simulink model "Sim_PMSMCtrl"  (R2025b)
settings: Solver=FixedStepAuto  StartTime=0.0  StopTime=0.1  RelTol=1e-3
values from neighbouring files (symbols this model uses):
  Par_Sim_cdSysTs = 5.0E-8    [Sim_PMSMCtrl.sldd]
undefined symbols (not defined in the file or in its folder): Par_Cpu_cfCoreFrc, Par_Cpu_cfTpwm
libraries: nesl_utility x14, fl_lib x8, ee_lib x5, mcbeeMathTransformLib x4, Lib_General x3, batteryecm_lib x1, Lib_PMSMCtrl x1
settings Model: DataDictionary=Sim_PMSMCtrl.sldd  SimulationMode=accelerator  Creator=62555  LastModifiedBy=62555
settings OptimizationCC: DefaultParameterBehavior=Inlined  UseDivisionForNetSlopeComputation=on  DefaultUnderspecifiedDataType=single  EnhancedBackFolding=on  PassReuseOutputArgsAs=Individual arguments  ZeroExternalMemoryAtStartup=off  ZeroInternalMemoryAtStartup=off  OptimizeBlockOrder=speed  DifferentSizesBufferReuse=on  OptimizationCustomize=off  EfficientTunableParamExpr=on
settings DebuggingCC: ParameterPrecisionLossMsg=none  ParameterTunabilityLossMsg=error
settings SFSimCC: MATLABDynamicMemAlloc=off
settings RTWCC: SystemTargetFile=ert.tlc  GenCodeOnly=on  TemplateMakefile=ert_default_tmf  GenerateReport=on  Toolchain=CMake  LaunchReport=on  GPUComputeCapability=3.5  Description=Embedded Coder
settings CodeAppCC: ForceParamTrailComments=on  IgnoreCustomStorageClasses=off  OperatorAnnotations=on  SimulinkDataObjDesc=on  SFDataObjDesc=on  InsertBlockDesc=on
settings ERTTargetCC: ERTCustomFileTemplate=example_file_process.tlc  DynamicArrayContainerType=coder::array  TargetLangStandard=C99 (ISO)  GenerateSampleERTMain=on

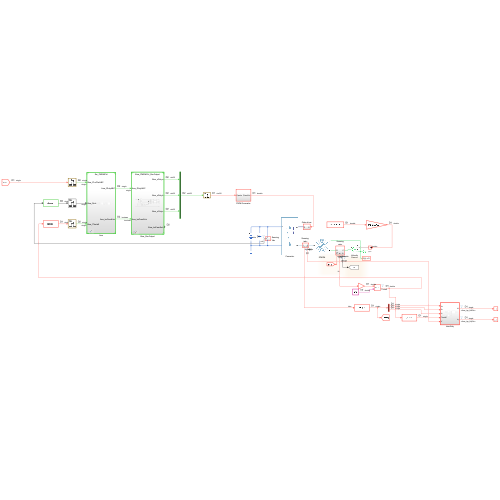
[thumbnail: Simulink's stored preview of the top-level diagram]
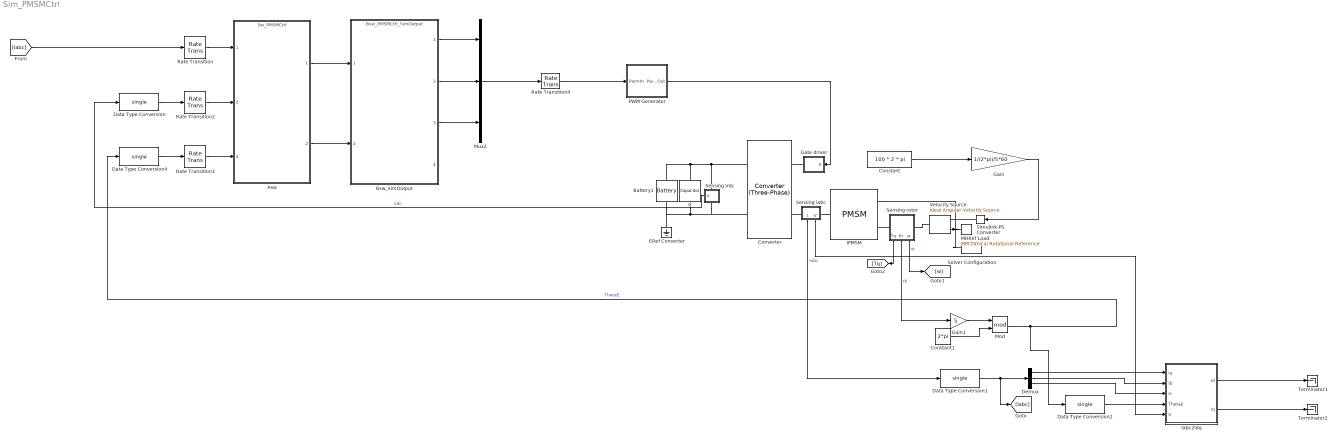
== system Sim_PMSMCtrl ==
  Asw : ModelReference  ModelNameDialog=Sw_PMSMCtrl.slx  SimulationMode=Normal  ModelReferenceVersion=6.16
  Battery1 : batteryecm_lib/Battery  Vnom=48 V  prm_dir=1  R1_dis=2 Ohm  R1_ch=2 Ohm  R1=0.001 Ohm  prm_AH=1  AH=300 hr*A  V1=V1 V  AH1=100 hr*A  prm_R2=1  R2=2000 Ohm  Tmeas=298.15 K  charge_measurement_port=simscape.enum.battery.enable.no  prm_dyn=1  Rp1=0.005 Ohm  tau1=30 s  Rp2=0.005 Ohm  tau2=30 s  Rp3=0.005 Ohm  tau3=30 s  Rp4=0.005 Ohm  tau4=30 s  Rp5=0.005 Ohm  tau5=30 s  prm_fade=1  N_fade=100  AH_fade=45 hr*A  R1_fade=2.02 Ohm  R1_ch_fade=2.02 Ohm  V1_fade=10.35 V  prm_age=1  prm_age_OCV=1  OCV_age=0.9  SOC_age=60  Tmeas_age=298.15 K  delta_time_age_vec=[0] d  temperature_age_vec=[273] K  OCV_scaling_age=2.2134e6  OCV_offset_age=1.632e6  temp_exp_age=0.515833569 V  t_exp_age=0.75  Vnom_T2=12 V  R1_T2=2.2 Ohm  R1_T2_dis=2.2 Ohm  R1_T2_ch=2.2 Ohm  V1_T2=11.4 V  R2_T2=2200 Ohm  Rp1_T2=0.005 Ohm  tau1_T2=30 s  Rp2_T2=0.005 Ohm  tau2_T2=30 s  Rp3_T2=0.005 Ohm  tau3_T2=30 s  Rp4_T2=0.005 Ohm  tau4_T2=30 s  Rp5_T2=0.005 Ohm  tau5_T2=30 s  Tmeas2=273.15 K  thermal_port=simscape.enum.thermaleffects.omit  thermal_mass=30000 J/K  i_specify=off  i_priority=None  i=0 A  i_nominal_specify=off  i_nominal_value=1  i_nominal_unit=A  v_specify=off  v_priority=None  v=0 V  v_nominal_specify=off  v_nominal_value=1  v_nominal_unit=V  charge_specify=on  charge_priority=High  charge=50 hr*A  charge_nominal_specify=off  charge_nominal_value=1  charge_nominal_unit=A*hr  num_cycles_specify=off  num_cycles_priority=High  num_cycles=0  num_cycles_nominal_specify=off  num_cycles_nominal_value=1  num_cycles_nominal_unit=1  temperature_specify=off  temperature_priority=High  temperature=298.15 K  temperature_nominal_specify=off  temperature_nominal_value=1  temperature_nominal_unit=K
  Bsw_SimOutput : ModelReference  ModelNameDialog=Bsw_PMSMCtrl_SimOutput.slx  SimulationMode=Normal  ModelReferenceVersion=6.3
  C : fl_lib/Electrical/Electrical Elements/Capacitor  c=5e-6 F  r=1e-6 Ohm  g=0 1/Ohm  i_specify=off  i_priority=None  i=0 A  i_nominal_specify=off  i_nominal_value=1  i_nominal_unit=A  v_specify=off  v_priority=None  v=0 V  v_nominal_specify=off  v_nominal_value=1  v_nominal_unit=V  vc_specify=on  vc_priority=None  vc=48 V  vc_nominal_specify=off  vc_nominal_value=1  vc_nominal_unit=V
  Constant : Constant  Value=100 * 2 * pi  SampleTime=-1
  Constant1 : Constant  Value=2*pi
  Converter : ee_lib/Semiconductors & Converters/Converters/Converter (Three-Phase)  port_option=ee.enum.threePhasePort.composite  fidelity_option=ee.enum.converters.fidelity.detailed  device_type=ee.enum.converters.switchingdevice.mosfet  showThermalPort=false  K=0  Vth=0.005 V  Vgt=1 V  Vgt_off=-1 V  Ih=1 A  Vf=0.005 V  Ron=0.001 Ohm  Rds=0.001 Ohm  Goff=1e-5 1/Ohm  Eon_scalar=22.86e-3 J  Eoff_scalar=17.14e-3 J  Eoff_natural_commutation=10e-3 J  Voff=300 V  Iout_scalar=600 A  onCurrentMeasDelay=0 s  useCurrentFromPreviousCycle=false  useVoltageFromPreviousCycle=false  diode_param=ee.enum.converters.protectiondiode.none  diode_Vf=0.8 V  diode_Ron=0.001 Ohm  diode_Goff=1e-5 1/Ohm  diode_C=50 nF  diode_iRM=-235 A  diode_iF=300 A  diode_idot=-50 A/us  diode_trr_param=1  diode_trr_factor=3  diode_trr=15 us  diode_Qrr=1.5e+3 s*uA  diode_rec_loss_model=ee.enum.diode.reverseRecoveryModel.fixed  diode_ErecVal=0 J  diode_scaleWithIandV=false  diode_ErecMat=zeros(2, 3) J  diode_TjrecVec=[298.15, 398.15] K  diode_IfrecVec=[.1, 1, 10] A  diode_IrecVal=10 A  diode_VrecVal=10 V  diode_tFilter=1 / 1000 / 100 s  thermal_network_parameterization=ee.enum.thermalNetworkTopology.external  Rth=[.08, .5] K/W  Rth_Cauer=[.08, .1, .5] K/W  Rth_Foster=[.08, .14, .22, .16] K/W  thermal_mass_parameterization=ee.enum.thermalNetwork.timeconstant  thermal_mass=[.01, .5] J/K  thermal_mass_Cauer=[.01, .1, .5] J/K  thermal_mass_Foster=[.001, .005, .05, .5] J/K  thermal_time_constant=[.001, .2] s  thermal_time_constant_Cauer=[.001, .1, .2] s  thermal_time_constant_Foster=[7e-05, .0007, .01, .08] s  thermal_mass_initial_temperatures=[25, 25] degC  thermal_mass_initial_temperatures_Cauer=[25, 25, 25] degC  junction_thermal_mass=0.01 J/K  Tvec_initial_Foster=[25, 25, 25, 25] degC  snubber_type=0  Cs=1e-7 F  Rs=0.1 Ohm  Vce_loss=[0, 150, 300] V
  Data Type Conversion{,1..2,4} (4 alike) : DataTypeConversion  OutDataTypeStr=single  SaturateOnIntegerOverflow=off  RndMeth=Floor
  Demux : Demux  Outputs=3
  ERef Converter : fl_lib/Electrical/Electrical Elements/Electrical Reference
  Gain : Gain  Gain=1/(2*pi)/5*60
  Gain1 : Gain  Gain=5
  Gate driver : Subsystem
  IPMSM : ee_lib/Electromechanical/Permanent Magnet/PMSM  port_option=ee.enum.threePhasePort.composite  winding_type=ee.enum.statorconnection.wye  machine_param=ee.enum.pmsm.parameterization.constant  nPolePairs=5  pmflux_param=ee.enum.pmflux.fluxlinkage  pm_flux_linkage=Par_Mtr_cfFlux Wb  torque_constant=0.18 N*m/A  back_emf_constant=0.18 V/(rad/s)  stator_param=ee.enum.statorparam.LdLqL0  Ld=Par_Mtr_cfLd H  Lq=Par_Mtr_cfLq H  idVec=[-200, 0, 200] A  iqVec=[-200, 0, 200] A  LdMatrix=0.0002 * ones(3, 3) H  LqMatrix=0.0002 * ones(3, 3) H  PmMatrix=0.1 * ones(3, 3) Wb  ktMatrix=0.18 * ones(3, 3) N*m/A  keMatrix=0.18 * ones(3, 3) V/(rad/s)  L0=L0 H  Ls=0.0002 H  Lm=0.00002 H  Ms=0.00002 H  Rs=Par_Mtr_cfRs Ohm  zero_sequence=ee.enum.park.zerosequence.exclude  axes_param=ee.enum.rotorangle.daxis  loss_param=ee.enum.ironloss.none  losses_oc=[0, 0, 0] W  losses_sc=[0, 0, 0] W  f_losses=60 Hz  Isc_losses=95 A  J=0 kg*m^2  lam=0 N*m/(rad/s)  i_d_specify=off  i_d_priority=None  i_d=0 A  i_d_nominal_specify=off  i_d_nominal_value=1  i_d_nominal_unit=A  i_q_specify=off  i_q_priority=None  i_q=0 A  i_q_nominal_specify=off  i_q_nominal_value=1  i_q_nominal_unit=A  torque_specify=off  torque_priority=None  torque=0 N*m  torque_nominal_specify=off  torque_nominal_value=1  torque_nominal_unit=N*m  angular_velocity_specify=on  angular_velocity_priority=None  angular_velocity=0 rad/s  angular_velocity_nominal_specify=off  angular_velocity_nominal_value=1  angular_velocity_nominal_unit=rpm  angular_position_specify=on  angular_position_priority=High  angular_position=0 rad  angular_position_nominal_specify=off  angular_position_nominal_value=1  angular_position_nominal_unit=deg  alpha=3.93e-3 1/K  alpha_flux=-0.001 1/K  Tmeas=298.15 K  stator_thermal_mass=100 J/K  rotor_thermal_mass=200 J/K  Rm_percent_rotor=90  Rd_percent_rotor=30  temperatureA_specify=off  temperatureA_priority=High  temperatureA=25 degC  temperatureA_nominal_specify=off  temperatureA_nominal_value=1  temperatureA_nominal_unit=degC  temperatureB_specify=off  temperatureB_priority=High  temperatureB=25 degC  temperatureB_nominal_specify=off  temperatureB_nominal_value=1  temperatureB_nominal_unit=degC  temperatureC_specify=off  temperatureC_priority=High  temperatureC=25 degC  temperatureC_nominal_specify=off  temperatureC_nominal_value=1  temperatureC_nominal_unit=degC  temperatureR_specify=off  temperatureR_priority=High  temperatureR=25 degC  temperatureR_nominal_specify=off  temperatureR_nominal_value=1  temperatureR_nominal_unit=degC
      settings: InternalSimscapePortConfiguration="{\"Bottom\":[],\"Left\":[{\"id\":\"N\",\"label\":\"~\",\"type\":\"foundation.electrical.three_phase\"}],\"Right\":[{\"id\":\"R\",\"label\":\"R\",\"type\":\"foundation.mechanical.rotational.rotational\"},{\"id\":\"C\",\"label\":\"C\",\"type\":\"foundation.mechanical.rotational.rotational\"}],\"Top\":[]}"
  Iabc2Idq : Subsystem  TreatAsAtomicUnit=on
      settings: RTWSystemCode=Nonreusable function  RTWFcnNameOpts=Use subsystem name  FunctionInterfaceSpec=Allow arguments (Optimized)
  MRRef Load : fl_lib/Mechanical/Rotational Elements/Mechanical Rotational Reference
  Mod : Math  Operator=mod
  Mux2 : Mux  Inputs=3
  PWM Generator : Subsystem
  Rate Transition : RateTransition  OutPortSampleTime=Par_Sw_cdTs
  Rate Transition1 : RateTransition  OutPortSampleTime=Par_Sw_cdTs
  Rate Transition2 : RateTransition  OutPortSampleTime=Par_Sw_cdTs
  Rate Transition4 : RateTransition  OutPortSampleTime=Par_Sim_cdSysTs
  Sensing Vdc : Subsystem
      settings: PortSchema="{\"entries\":[{\"content\":{\"sides\":[{\"content\":{\"connectorIds\":[\"LConn1\"]},\"type\":\"ConnectorPlacement.EquallySpacedRectSide\",\"uuid\":\"bc3757cc-4537-444e-89af-7b7d8c8c1fa7\"},{\"content\":{\"connectorIds\":[\"RConn1\"],\"side\":\"RIGHT\"},\"type\":\"ConnectorPlacement.EquallySpacedRectSide\",\"uuid\":\"908bf4c4-26f6-4d8a-bcf8-68236027f5f8\"},{\"content\":{\"connectorIds\":[\"Out1\"],\"side\":\"TOP\"},\"type\":\"ConnectorPlacement.EquallySpacedRectSide\",\"uuid\":\"33f228db-ba47-4718-96dc-a72de309ae8c\"},{\"content\":{\"connectorIds\":[],\"side\":\"BOTTOM\"},\"type\":\"ConnectorPlacement.EquallySpacedRectSide\",\"uuid\":\"d9b66c7e-0954-4c47-8bcc-77bf13ff573c\"}]},\"type\":\"ConnectorPlacement.EquallySpacedConnector\",\"uuid\":\"345f3578-0572-4e64-b2f3-84728129a12d\"}],\"packageUris\":[\"http://schema.mathworks.com/mf0/Connector/R2020b\"],\"version\":\"1.0\"}"
  Sensing rotor : Subsystem
      settings: PortSchema="{\"entries\":[{\"content\":{\"sides\":[{\"content\":{\"connectorIds\":[\"LConn1\"]},\"type\":\"ConnectorPlacement.EquallySpacedRectSide\",\"uuid\":\"bc3757cc-4537-444e-89af-7b7d8c8c1fa7\"},{\"content\":{\"connectorIds\":[\"RConn1\"],\"side\":\"RIGHT\"},\"type\":\"ConnectorPlacement.EquallySpacedRectSide\",\"uuid\":\"908bf4c4-26f6-4d8a-bcf8-68236027f5f8\"},{\"content\":{\"connectorIds\":[],\"side\":\"TOP\"},\"type\":\"ConnectorPlacement.EquallySpacedRectSide\",\"uuid\":\"33f228db-ba47-4718-96dc-a72de309ae8c\"},{\"content\":{\"connectorIds\":[\"Out1\",\"Out2\",\"Out3\"],\"side\":\"BOTTOM\"},\"type\":\"ConnectorPlacement.EquallySpacedRectSide\",\"uuid\":\"5b763560-fcc9-460b-9ba7-46235112184c\"}]},\"type\":\"ConnectorPlacement.EquallySpacedConnector\",\"uuid\":\"345f3578-0572-4e64-b2f3-84728129a12d\"}],\"packageUris\":[\"http://schema.mathworks.com/mf0/Connector/R2020b\"],\"version\":\"1.0\"}"
  Sensing iabc : Subsystem
      settings: PortSchema="{\"entries\":[{\"content\":{\"sides\":[{\"content\":{\"connectorIds\":[\"LConn1\"]},\"type\":\"ConnectorPlacement.EquallySpacedRectSide\",\"uuid\":\"bc3757cc-4537-444e-89af-7b7d8c8c1fa7\"},{\"content\":{\"connectorIds\":[\"RConn1\"],\"side\":\"RIGHT\"},\"type\":\"ConnectorPlacement.EquallySpacedRectSide\",\"uuid\":\"908bf4c4-26f6-4d8a-bcf8-68236027f5f8\"},{\"content\":{\"side\":\"TOP\"},\"type\":\"ConnectorPlacement.EquallySpacedRectSide\",\"uuid\":\"33f228db-ba47-4718-96dc-a72de309ae8c\"},{\"content\":{\"connectorIds\":[\"Out1\",\"Out2\"],\"side\":\"BOTTOM\"},\"type\":\"ConnectorPlacement.EquallySpacedRectSide\",\"uuid\":\"3b1d40a5-3c80-431c-8111-df754e0c502b\"}]},\"type\":\"ConnectorPlacement.EquallySpacedConnector\",\"uuid\":\"345f3578-0572-4e64-b2f3-84728129a12d\"}],\"packageUris\":[\"http://schema.mathworks.com/mf0/Connector/R2020b\"],\"version\":\"1.0\"}"
  Simulink-PS Converter : nesl_utility/Simulink-PS Converter  PhysicalDomain=network_engine_domain  SubClassName=ps_input  LeftPortType=input  RightPortType=output  PseudoPeriodic=off  Frequencies=[]  NoiseDistribution=none  NoiseParameters=[]  Unit=rpm  AffineConversion=off  FilteringAndDerivatives=zero  SimscapeFilterOrder=1  InputFilterTimeConstant=0.001  UdotUserProvided=1
  Solver Configuration : nesl_utility/Solver Configuration  PhysicalDomain=network_engine_domain  SubClassName=solver  LeftPortType=input  RightPortType=generic  Tones=[]  Harmonics=[]  SimulateNoise=off  Profile=off  UseLocalSampling=off  EnableSwitchedLinearOptims=on  FrequencyDomain=off  UseCCode=off  RelTol=0.001  AbsTol=1e-06  MinStep=1e-09  ToWorkspace=off  RevertToSquareIcSolve=off  NumHomotopyIterations=100  PhasorMode=off  PhasorModeNumHarmonics=1  ConsistencySolver=NEWTON_FTOL  IndexReductionMethod=DerivativeReplacement  DoDC=off  ResidualTolerance=1e-9  ConsistencyTolSource=GLOBAL  ConsistencyAbsTol=0.001  ConsistencyRelTol=0.001  ConsistencyTolFactor=0.001  UseLocalSolver=on  LocalSolverChoice=NE_BACKWARD_EULER_ADVANCER  ResolveIndetEquations=on  FunctionEvalNumThread=1  LocalSolverSampleTime=Par_Sim_cdSysTs  DoFixedCost=on  MaxNonlinIter=5  MaxModeIter=2  ComputeImpulses=off  ImpulseIterations=2  LinearAlgebra=auto  LinearAlgebraNumThread=0  EquationFormulation=NE_TIME_EF  DelaysMemoryBudget=1024  AutomaticFiltering=on  FilteringTimeConstant=0.001  PartitionStorageMethod=AS_NEEDED  PartitionMemoryBudget=1024  PartitionMethod=FAST  MultibodyUseLocalSolver=off  MultibodyLocalSolverChoice=ODE1  MultibodyLocalSolverSampleTime=0.001
  Terminator1 : Terminator
  Terminator2 : Terminator
  Velocity Source : fl_lib/Mechanical/Mechanical Sources/Ideal Angular Velocity Source
  wires:
  Rate Transition4/1 -> PWM Generator/1(PwmIn)
  Mux2/1 -> Rate Transition4/1
  Data Type Conversion4/1 -> Rate Transition1/1
  Data Type Conversion/1 -> Rate Transition2/1
  Asw/1 -> Bsw_SimOutput/1
  Bsw_SimOutput/1 -> Mux2/1
  Bsw_SimOutput/2 -> Mux2/2
  Bsw_SimOutput/3 -> Mux2/3
  Sensing Vdc/1(V) -> Data Type Conversion/1  "vdc"
  Constant/1 -> Gain/1
  Sensing iabc/1(I) -> Data Type Conversion1/1  "Iabc"
  PWM Generator/1(PwmOut) -> Gate driver/1(S)
  Sensing rotor/2(th) -> Gain1/1  "th"
  Sensing rotor/1(Tq) -> [Tq]
  Gain/1 -> Simulink-PS Converter/1
  Gain1/1 -> Mod/1
  Constant1/1 -> Mod/2
  Mod/1 -> Data Type Conversion4/1, Data Type Conversion2/1  "ThetaE"
  Demux/1 -> Iabc2Idq/1(Ia)
  Demux/2 -> Iabc2Idq/2(Ib)
  Demux/3 -> Iabc2Idq/3(Ic)
  Iabc2Idq/1(Id) -> Terminator1/1
  Iabc2Idq/2(Iq) -> Terminator2/1
  Data Type Conversion1/1 -> [Iabc], Demux/1
  Data Type Conversion2/1 -> Iabc2Idq/4(ThetaE)
  Sensing iabc/2(V) -> Iabc2Idq/5(V)
  [Iabc] -> Rate Transition/1
  Asw/2 -> Bsw_SimOutput/2
  Rate Transition/1 -> Asw/1
  Rate Transition1/1 -> Asw/3
  Sensing rotor/3(w) -> [w]  "w"
  Rate Transition2/1 -> Asw/2
  connections:
  C/LConn1 -- Converter/RConn1 -- Sensing Vdc/LConn1 -- Battery1/LConn1
  MRRef Load/LConn1 -- IPMSM/RConn2 -- Velocity Source/RConn2 -- Solver Configuration/RConn1
  C/RConn1 -- Converter/RConn2 -- Sensing Vdc/RConn1 -- Battery1/RConn1 -- ERef Converter/LConn1
  Simulink-PS Converter/RConn1 -- Velocity Source/RConn1
  Sensing iabc/LConn1 -- Converter/LConn2
  Sensing iabc/RConn1 -- IPMSM/LConn1
  Gate driver/RConn1 -- Converter/LConn1
  Sensing rotor/LConn1 -- IPMSM/RConn1
  Sensing rotor/RConn1 -- Velocity Source/LConn1

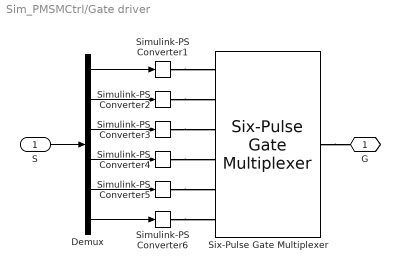
== system Sim_PMSMCtrl/Gate driver ==
  S : Inport
  Demux : Demux  Outputs=6
  Simulink-PS Converter{1..6} (6 alike) : nesl_utility/Simulink-PS Converter  PhysicalDomain=network_engine_domain  SubClassName=ps_input  LeftPortType=input  RightPortType=output  PseudoPeriodic=off  Frequencies=[]  NoiseDistribution=none  NoiseParameters=[]  Unit=1  AffineConversion=off  FilteringAndDerivatives=zero  SimscapeFilterOrder=1  InputFilterTimeConstant=0.001  UdotUserProvided=1
  Six-Pulse Gate Multiplexer : ee_lib/Semiconductors & Converters/Converters/Six-Pulse Gate Multiplexer  port_option=ee.enum.controlport.ps
  G : PMIOPort  Side=Right
  wires:
  Demux/1 -> Simulink-PS Converter1/1
  S/1 -> Demux/1
  Demux/5 -> Simulink-PS Converter5/1
  Demux/6 -> Simulink-PS Converter6/1
  Demux/4 -> Simulink-PS Converter4/1
  Demux/3 -> Simulink-PS Converter3/1
  Demux/2 -> Simulink-PS Converter2/1
  connections:
  Six-Pulse Gate Multiplexer/RConn1 -- G/RConn1
  Simulink-PS Converter1/RConn1 -- Six-Pulse Gate Multiplexer/LConn1
  Simulink-PS Converter5/RConn1 -- Six-Pulse Gate Multiplexer/LConn5
  Simulink-PS Converter6/RConn1 -- Six-Pulse Gate Multiplexer/LConn6
  Simulink-PS Converter2/RConn1 -- Six-Pulse Gate Multiplexer/LConn2
  Simulink-PS Converter3/RConn1 -- Six-Pulse Gate Multiplexer/LConn3
  Simulink-PS Converter4/RConn1 -- Six-Pulse Gate Multiplexer/LConn4

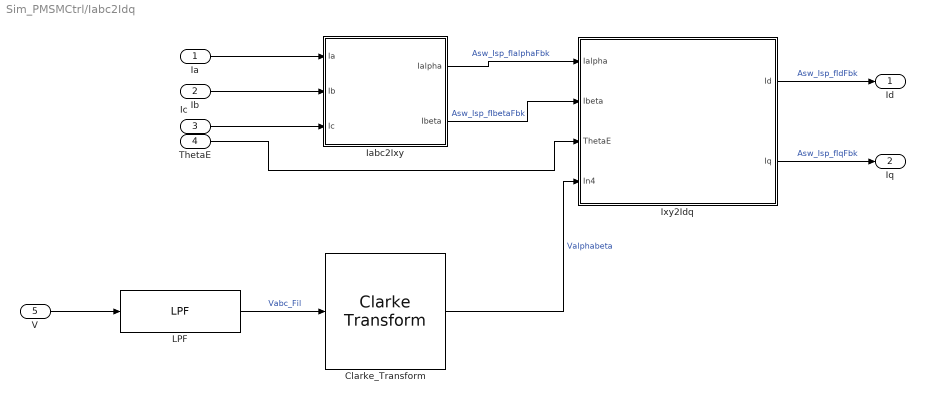
== system Sim_PMSMCtrl/Iabc2Idq ==
  Ia : Inport
  Ib : Inport  Port=2
  Ic : Inport  Port=3
  ThetaE : Inport  Port=4
  V : Inport  Port=5
  Clarke_Transform : mcbeeMathTransformLib/Clarke Transform  VariantControl=Variant2  PowerInvariant=off  UseWithEmbedded=on  PhaseInput=Three inputs
  Iabc2Ixy : Subsystem  TreatAsAtomicUnit=on
      settings: RTWSystemCode=Nonreusable function  RTWFcnNameOpts=Use subsystem name  FunctionInterfaceSpec=Allow arguments (Optimized)
  Ixy2Idq : Subsystem  TreatAsAtomicUnit=on
      settings: RTWSystemCode=Nonreusable function  RTWFcnNameOpts=Use subsystem name  FunctionInterfaceSpec=Allow arguments (Optimized)
  LPF : Lib_General/LPF  fc=1e3  Initial_condition=0  ModType=Tustin
      settings: SourceProductName=Lib_General
      settings: AttributesFormatString=|
      | fc = %<fc>
      | DisMod = %<ModType>
  Id : Outport
  Iq : Outport  Port=2
  wires:
  Ixy2Idq/2(Iq) -> Iq/1  "Asw_Isp_fIqFbk"
  Ia/1 -> Iabc2Ixy/1(Ia)
  ThetaE/1 -> Ixy2Idq/3(ThetaE)
  Ic/1 -> Iabc2Ixy/3(Ic)
  Ixy2Idq/1(Id) -> Id/1  "Asw_Isp_fIdFbk"
  Ib/1 -> Iabc2Ixy/2(Ib)
  Iabc2Ixy/2(Ibeta) -> Ixy2Idq/2(Ibeta)  "Asw_Isp_fIbetaFbk"
  Iabc2Ixy/1(Ialpha) -> Ixy2Idq/1(Ialpha)  "Asw_Isp_fIalphaFbk"
  Clarke_Transform/1 -> Ixy2Idq/4(In4)  "Valphabeta"
  V/1 -> LPF/1
  LPF/1 -> Clarke_Transform/1  "Vabc_Fil"

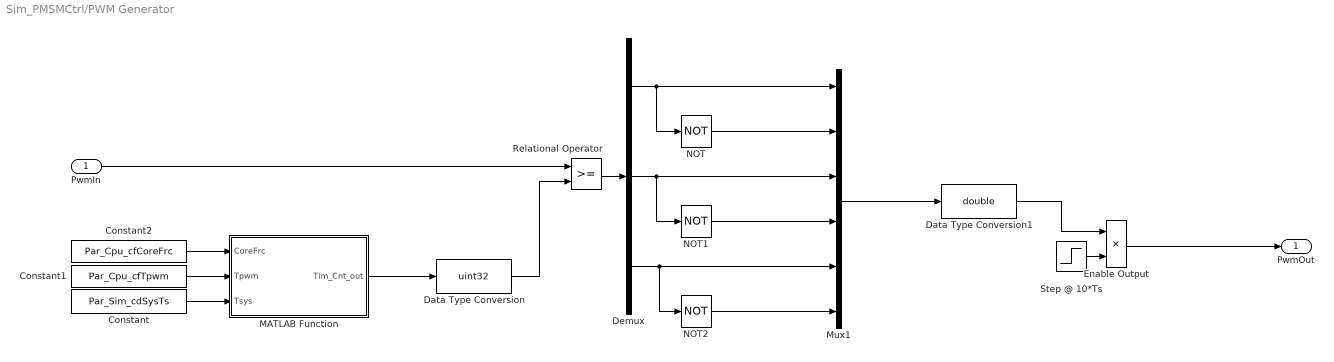
== system Sim_PMSMCtrl/PWM Generator ==
  PwmIn : Inport
  Constant : Constant  Value=Par_Sim_cdSysTs  OutDataTypeStr=double  SampleTime=-1
  Constant1 : Constant  Value=Par_Cpu_cfTpwm  OutDataTypeStr=double  SampleTime=-1
  Constant2 : Constant  Value=Par_Cpu_cfCoreFrc  OutDataTypeStr=double  SampleTime=-1
  Data Type Conversion : DataTypeConversion  OutDataTypeStr=uint32  SaturateOnIntegerOverflow=off  RndMeth=Floor
  Data Type Conversion1 : DataTypeConversion  OutDataTypeStr=double  SaturateOnIntegerOverflow=off  RndMeth=Floor
  Demux : Demux  Outputs=3
  Enable Output : Product
  MATLAB Function : MATLAB Function  TreatAsAtomicUnit=on
  Mux1 : Mux  Inputs=6
  NOT : Logic  Operator=NOT  IconShape=distinctive  AllPortsSameDT=off  OutDataTypeStr=boolean
  NOT1 : Logic  Operator=NOT  IconShape=distinctive  AllPortsSameDT=off  OutDataTypeStr=boolean
  NOT2 : Logic  Operator=NOT  IconShape=distinctive  AllPortsSameDT=off  OutDataTypeStr=boolean
  Relational Operator : RelationalOperator  OutDataTypeStr=boolean  RndMeth=Simplest  InputSameDT=off
  Step @ 10*Ts : Step  Time=0.00050  SampleTime=Par_Sim_cdSysTs
  PwmOut : Outport
  wires:
  Demux/1 -> Mux1/1, NOT/1
  Demux/3 -> NOT2/1, Mux1/5
  Demux/2 -> NOT1/1, Mux1/3
  NOT2/1 -> Mux1/6
  NOT/1 -> Mux1/2
  MATLAB Function/1(Tim_Cnt_out) -> Data Type Conversion/1
  NOT1/1 -> Mux1/4
  Relational Operator/1 -> Demux/1
  PwmIn/1 -> Relational Operator/1
  Constant/1 -> MATLAB Function/3(Tsys)
  Constant1/1 -> MATLAB Function/2(Tpwm)
  Constant2/1 -> MATLAB Function/1(CoreFrc)
  Data Type Conversion/1 -> Relational Operator/2
  Mux1/1 -> Data Type Conversion1/1
  Data Type Conversion1/1 -> Enable Output/1
  Step @ 10*Ts/1 -> Enable Output/2
  Enable Output/1 -> PwmOut/1

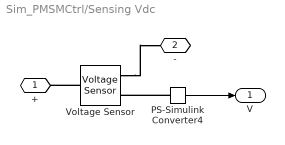
== system Sim_PMSMCtrl/Sensing Vdc ==
  PS-Simulink Converter4 : nesl_utility/PS-Simulink Converter  PhysicalDomain=network_engine_domain  SubClassName=ps_output  LeftPortType=input  RightPortType=output  PseudoPeriodic=off  Frequencies=[]  VectorFormat=1-D array  Unit=V  AffineConversion=off
  Voltage Sensor : fl_lib/Electrical/Electrical Sensors/Voltage Sensor
  + : PMIOPort  Side=Left
  - : PMIOPort  Port=2  Side=Right
  V : Outport
  wires:
  PS-Simulink Converter4/1 -> V/1
  connections:
  Voltage Sensor/LConn1 -- +/RConn1
  Voltage Sensor/RConn2 -- -/RConn1
  PS-Simulink Converter4/LConn1 -- Voltage Sensor/RConn1

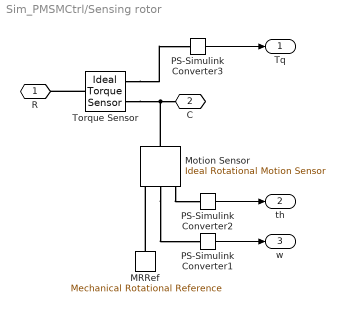
== system Sim_PMSMCtrl/Sensing rotor ==
  MRRef : fl_lib/Mechanical/Rotational Elements/Mechanical Rotational Reference
  Motion Sensor : fl_lib/Mechanical/Mechanical Sensors/Ideal Rotational Motion Sensor  reference=foundation.enum.MeasurementReference.difference  acceleration_port=false  velocity_port=true  position_port=true  wrap_angle=simscape.enum.onoff.off  offset=0 deg
  PS-Simulink Converter1 : nesl_utility/PS-Simulink Converter  PhysicalDomain=network_engine_domain  SubClassName=ps_output  LeftPortType=input  RightPortType=output  PseudoPeriodic=off  Frequencies=[]  VectorFormat=1-D array  Unit=rad/s  AffineConversion=off
  PS-Simulink Converter2 : nesl_utility/PS-Simulink Converter  PhysicalDomain=network_engine_domain  SubClassName=ps_output  LeftPortType=input  RightPortType=output  PseudoPeriodic=off  Frequencies=[]  VectorFormat=1-D array  Unit=rad  AffineConversion=off
  PS-Simulink Converter3 : nesl_utility/PS-Simulink Converter  PhysicalDomain=network_engine_domain  SubClassName=ps_output  LeftPortType=input  RightPortType=output  PseudoPeriodic=off  Frequencies=[]  VectorFormat=1-D array  Unit=N*m  AffineConversion=off
  Torque Sensor : fl_lib/Mechanical/Mechanical Sensors/Ideal Torque Sensor
  R : PMIOPort  Side=Left
  C : PMIOPort  Port=2  Side=Right
  Tq : Outport
  th : Outport  Port=2
  w : Outport  Port=3
  wires:
  PS-Simulink Converter3/1 -> Tq/1
  PS-Simulink Converter2/1 -> th/1
  PS-Simulink Converter1/1 -> w/1
  connections:
  Torque Sensor/RConn1 -- Motion Sensor/LConn1 -- C/RConn1
  Torque Sensor/RConn2 -- PS-Simulink Converter3/LConn1
  Torque Sensor/LConn1 -- R/RConn1
  Motion Sensor/RConn2 -- PS-Simulink Converter1/LConn1
  MRRef/LConn1 -- Motion Sensor/RConn1
  Motion Sensor/RConn3 -- PS-Simulink Converter2/LConn1

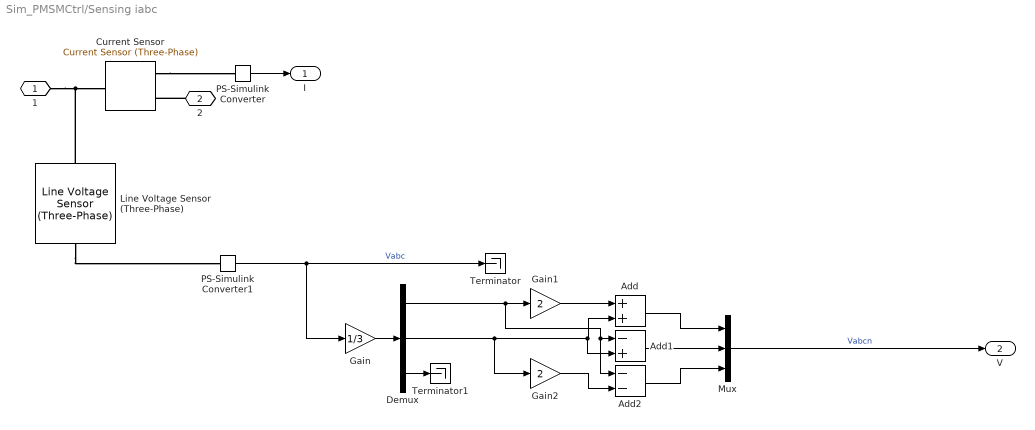
== system Sim_PMSMCtrl/Sensing iabc ==
  Add : Sum
  Add1 : Sum  Inputs=-+
  Add2 : Sum  Inputs=--
  Current Sensor : ee_lib/Sensors & Transducers/Current Sensor (Three-Phase)
  Demux : Demux  Outputs=3
  Gain : Gain  Gain=1/3
  Gain1 : Gain  Gain=2
  Gain2 : Gain  Gain=2
  Line Voltage Sensor (Three-Phase) : ee_lib/Sensors & Transducers/Line Voltage Sensor (Three-Phase)
  Mux : Mux  Inputs=3
  PS-Simulink Converter : nesl_utility/PS-Simulink Converter  PhysicalDomain=network_engine_domain  SubClassName=ps_output  LeftPortType=input  RightPortType=output  PseudoPeriodic=off  Frequencies=[]  VectorFormat=1-D array  Unit=A  AffineConversion=off
  PS-Simulink Converter1 : nesl_utility/PS-Simulink Converter  PhysicalDomain=network_engine_domain  SubClassName=ps_output  LeftPortType=input  RightPortType=output  PseudoPeriodic=off  Frequencies=[]  VectorFormat=1-D array  Unit=V  AffineConversion=off
  Terminator : Terminator
  Terminator1 : Terminator
  1 : PMIOPort  Side=Left
  2 : PMIOPort  Port=2  Side=Right
  I : Outport
  V : Outport  Port=2
  wires:
  PS-Simulink Converter/1 -> I/1
  PS-Simulink Converter1/1 -> Terminator/1, Gain/1  "Vabc"
  Gain/1 -> Demux/1
  Gain1/1 -> Add/1
  Demux/2 -> Gain2/1, Add1/2, Add/2
  Gain2/1 -> Add2/2
  Demux/1 -> Add2/1, Add1/1, Gain1/1
  Add1/1 -> Mux/2
  Add/1 -> Mux/1
  Add2/1 -> Mux/3
  Mux/1 -> V/1  "Vabcn"
  Demux/3 -> Terminator1/1
  connections:
  1/RConn1 -- Line Voltage Sensor (Three-Phase)/LConn1 -- Current Sensor/LConn1
  2/RConn1 -- Current Sensor/RConn2
  Current Sensor/RConn1 -- PS-Simulink Converter/LConn1
  Line Voltage Sensor (Three-Phase)/RConn1 -- PS-Simulink Converter1/LConn1

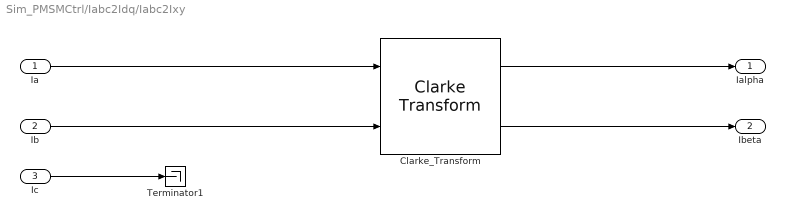
== system Sim_PMSMCtrl/Iabc2Idq/Iabc2Ixy ==
  Ia : Inport
  Ib : Inport  Port=2
  Ic : Inport  Port=3
  Clarke_Transform : mcbeeMathTransformLib/Clarke Transform  VariantControl=Variant2  PowerInvariant=off  UseWithEmbedded=on  PhaseInput=Two inputs
  Terminator1 : Terminator
  Ialpha : Outport
  Ibeta : Outport  Port=2
  wires:
  Ib/1 -> Clarke_Transform/2
  Ia/1 -> Clarke_Transform/1
  Ic/1 -> Terminator1/1
  Clarke_Transform/2 -> Ibeta/1
  Clarke_Transform/1 -> Ialpha/1

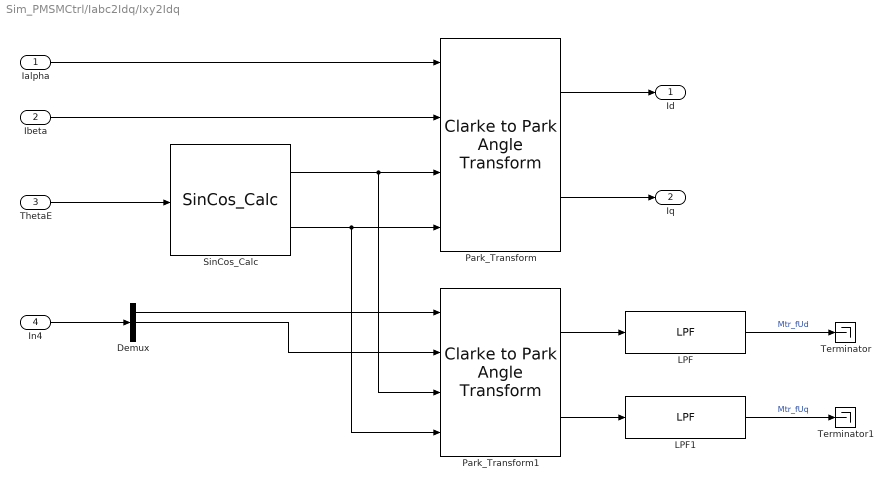
== system Sim_PMSMCtrl/Iabc2Idq/Ixy2Idq ==
  Ialpha : Inport
  Ibeta : Inport  Port=2
  ThetaE : Inport  Port=3
  In4 : Inport  Port=4
  Demux : Demux  Outputs=3
  LPF : Lib_General/LPF  fc=1e2  Initial_condition=0  ModType=Tustin
      settings: SourceProductName=Lib_General
      settings: AttributesFormatString=|
      | fc = %<fc>
      | DisMod = %<ModType>
  LPF1 : Lib_General/LPF  fc=1e2  Initial_condition=0  ModType=Tustin
      settings: SourceProductName=Lib_General
      settings: AttributesFormatString=|
      | fc = %<fc>
      | DisMod = %<ModType>
  Park_Transform : mcbeeMathTransformLib/Clarke to Park Angle Transform  AxisAlignment=D-axis  UseWithEmbedded=on  PhaseInput=Two inputs  ThetaInput=Sine and Cosine electrical position  AngleInput=Per-unit  N_points=1024
  Park_Transform1 : mcbeeMathTransformLib/Clarke to Park Angle Transform  AxisAlignment=D-axis  UseWithEmbedded=on  PhaseInput=Two inputs  ThetaInput=Sine and Cosine electrical position  AngleInput=Per-unit  N_points=1024
  SinCos_Calc : Lib_PMSMCtrl/SinCos_Calc
      settings: SourceProductName=Lib_PMSMCtrl
  Terminator : Terminator
  Terminator1 : Terminator
  Id : Outport
  Iq : Outport  Port=2
  wires:
  Ibeta/1 -> Park_Transform/2
  ThetaE/1 -> SinCos_Calc/1
  SinCos_Calc/2 -> Park_Transform1/4, Park_Transform/4
  Park_Transform/1 -> Id/1
  SinCos_Calc/1 -> Park_Transform1/3, Park_Transform/3
  Park_Transform/2 -> Iq/1
  Ialpha/1 -> Park_Transform/1
  In4/1 -> Demux/1
  Demux/1 -> Park_Transform1/1
  Demux/2 -> Park_Transform1/2
  Park_Transform1/1 -> LPF/1
  Park_Transform1/2 -> LPF1/1
  LPF/1 -> Terminator/1  "Mtr_fUd"
  LPF1/1 -> Terminator1/1  "Mtr_fUq"

== matlab function Sim_PMSMCtrl/PWM Generator/MATLAB Function ==
  data: CoreFrc input; Tim_Cnt_out output; Tpwm input; Tsys input
function Tim_Cnt_out = fcn(CoreFrc, Tpwm, Tsys)

  persistent Tim_Cnt;
  persistent Cnt_Flag;

  if isempty(Tim_Cnt)
    Tim_Cnt = double(0);
    Cnt_Flag = double(1);
  else

    Cnt_Lim = CoreFrc * Tpwm / 2;
    
    Tim_Cnt = Tim_Cnt + CoreFrc * Tsys * Cnt_Flag;
    
    if Cnt_Flag > 0 
      if Tim_Cnt > Cnt_Lim
        Tim_Cnt = 2 * Cnt_Lim - Tim_Cnt;
        Cnt_Flag = -1;
      end
    else
      if Tim_Cnt < 0
        Tim_Cnt = -Tim_Cnt;
        Cnt_Flag = 1;
      end
    end
  end
  Tim_Cnt_out = Tim_Cnt;
end
